simulink model "SMC_control"  (R2025b)
settings: Solver=ode4  StartTime=0.0  StopTime=50  FixedStep=1e-3  RelTol=1e-3
settings Model: Creator=feder  LastModifiedBy=feder

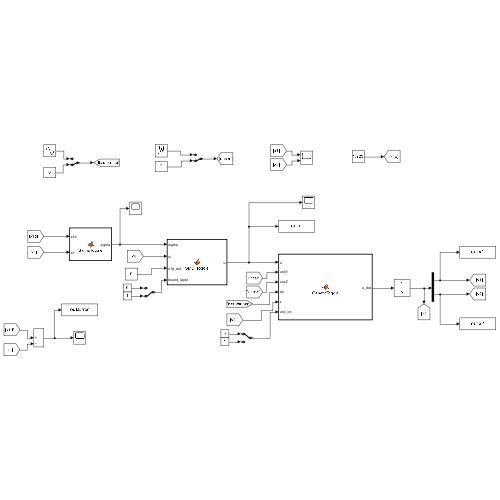
[thumbnail: Simulink's stored preview of the top-level diagram]
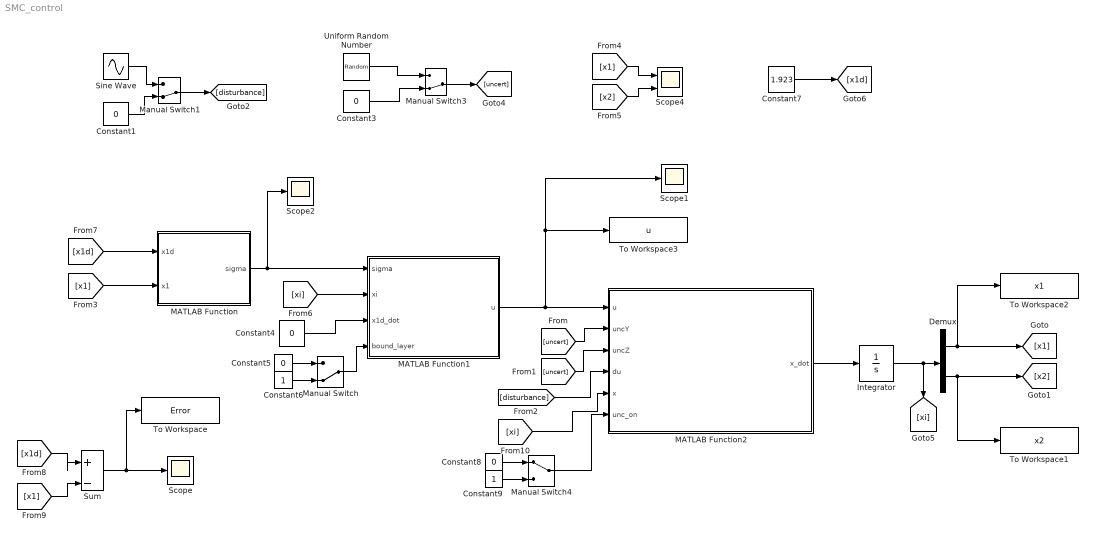
== system SMC_control ==
  Constant{1,3..5,8} (5 alike) : Constant  Value=0
  Constant6 : Constant
  Constant7 : Constant  Value=1.923
  Constant9 : Constant
  Demux : Demux  Outputs=2
  Integrator : Integrator  InitialCondition=[0.127;7.872]
  MATLAB Function : MATLAB Function  TreatAsAtomicUnit=on
  MATLAB Function1 : MATLAB Function  TreatAsAtomicUnit=on
  MATLAB Function2 : MATLAB Function  TreatAsAtomicUnit=on
  Manual Switch : ManualSwitch  CurrentSetting=0
  Manual Switch1 : ManualSwitch  CurrentSetting=0
  Manual Switch3 : ManualSwitch  CurrentSetting=0
  Manual Switch4 : ManualSwitch
  Scope : Scope
      settings: ActiveDisplayYMinimum=-16.327863972090057  ActiveDisplayYMaximum=16.683930684384531
  Scope1 : Scope
      settings: ActiveDisplayYMinimum=-112.46692384419836  ActiveDisplayYMaximum=360.72714778505906
  Scope2 : Scope
      settings: ActiveDisplayYMinimum=-16.118367270297529  ActiveDisplayYMaximum=10.830983390912735  DataLoggingVariableName=ScopeData2
  Scope4 : Scope  NumInputPorts=2
      settings: ActiveDisplayYMinimum=-1.6651704978189028  ActiveDisplayYMaximum=4.1664336792762047  DataLoggingVariableName=ScopeData4
  Sine Wave : Sin  Frequency=2*pi  SampleTime=0
  Sum : Sum  Inputs=|+-
  To Workspace : ToWorkspace  VariableName=Error  SaveFormat=Timeseries  SampleTime=-1
  To Workspace1 : ToWorkspace  VariableName=x2  SaveFormat=Timeseries  SampleTime=-1
  To Workspace2 : ToWorkspace  VariableName=x1  SaveFormat=Timeseries  SampleTime=-1
  To Workspace3 : ToWorkspace  VariableName=u  SaveFormat=Timeseries  SampleTime=-1
  Uniform Random Number : UniformRandomNumber  Minimum=-0.2  Maximum=0.2  SampleTime=1e6  VectorParams1D=off
  wires:
  [x1] -> Scope4/1
  [x2] -> Scope4/2
  Uniform Random Number/1 -> Manual Switch3/1
  Manual Switch3/1 -> [uncert]
  Manual Switch1/1 -> [disturbance]
  Constant3/1 -> Manual Switch3/2
  MATLAB Function/1(sigma) -> Scope2/1, MATLAB Function1/1(sigma)
  [uncert] -> MATLAB Function2/2(uncY)
  [disturbance] -> MATLAB Function2/4(du)
  Constant4/1 -> MATLAB Function1/3(x1d_dot)
  MATLAB Function2/1(x_dot) -> Integrator/1
  Demux/1 -> To Workspace2/1, [x1]
  Demux/2 -> [x2], To Workspace1/1
  Integrator/1 -> Demux/1, [xi]
  [xi] -> MATLAB Function1/2(xi)
  Constant5/1 -> Manual Switch/1
  Constant6/1 -> Manual Switch/2
  Manual Switch/1 -> MATLAB Function1/4(bound_layer)
  Constant7/1 -> [x1d]
  [x1d] -> MATLAB Function/1(x1d)
  [x1d] -> Sum/1
  [x1] -> Sum/2
  Sum/1 -> To Workspace/1, Scope/1
  Constant8/1 -> Manual Switch4/1
  Constant9/1 -> Manual Switch4/2
  Manual Switch4/1 -> MATLAB Function2/6(unc_on)
  [xi] -> MATLAB Function2/5(x)
  MATLAB Function1/1(u) -> MATLAB Function2/1(u), Scope1/1, To Workspace3/1
  [x1] -> MATLAB Function/2(x1)
  Constant1/1 -> Manual Switch1/2
  [uncert] -> MATLAB Function2/3(uncZ)
  Sine Wave/1 -> Manual Switch1/1

== matlab function SMC_control/MATLAB Function1 ==
  data: sigma input; u output; xi input; x1d_dot input; bound_layer input
function u = SMC_Toggle(sigma, xi, x1d_dot, bound_layer)

x1 = xi(1);
x2 = xi(2);

alphaY_nom = 10;     
betaY      = 0.25;
betaZ      = 0.25;


p1      = 9;        % 9 caso nominale
k       = 7;          % 3 caso nominale
epsilon = 0.01;      % 0.5 caso nominale pero va bene anche direttamente 0.01


D  = 1 + betaY/(1 + x2^2) + betaZ/(1 + x1^2);
g1 = 1/((1 + x2^2)*D);                         % first component of g(x)
f1 = alphaY_nom/((1 + x2^2)*D) - x1;           % first component of f(x)


Lie_der_f_sigma = p1*(f1 - x1d_dot);           % L_f sigma + partial_t sigma
Lie_der_g_sigma = p1*g1;                       % L_g sigma


if bound_layer
    if sigma > epsilon
        sw = 1;
    elseif sigma < -epsilon
        sw = -1;
    else
        sw = tanh(sigma/epsilon);              
    end
else
    sw = sign(sigma);
end

u = -(Lie_der_f_sigma + k*sw)/Lie_der_g_sigma;

end

% % ---- Control law (Raw) ----
% u_raw = -(Lie_der_f_sigma + k*sw)/Lie_der_g_sigma;
% 
% % ---- Input Saturation [-10, +30] ----
% % 1. min(u, 30)  -> Se u > 30, diventa 30.
% % 2. max(..., -10) -> Se il risultato è < -10, diventa -10.
% u = max(-10, min(u_raw, 30));
% 
% end

== matlab function SMC_control/MATLAB Function ==
  data: x1d input; x1 input; sigma output
function sigma = SigmaToggle(x1d, x1)
p1 = 9;              
sigma = p1*(x1 - x1d);
end

== matlab function SMC_control/MATLAB Function2 ==
  data: u input; uncY input; uncZ input; du input; x input; x_dot output; unc_on input
function x_dot = GeneticToggle(u, uncY, uncZ, du,x,unc_on)
alphaY_nom = 10;
alphaZ_nom = 10;
betaY_nom  = 0.25;
betaZ_nom  = 0.25;
gammaY     = 1;
gammaZ     = 1;
KY         = 1;
KZ         = 1;
n          = 2;

x1 = x(1);
x2 = x(2);


if unc_on
    alphaY_eff = alphaY_nom*(1 + uncY);
    alphaZ_eff = alphaZ_nom*(1 + uncZ);
    betaY = betaY_nom;  
    betaZ = betaZ_nom;
else
    alphaY_eff = alphaY_nom;
    alphaZ_eff = alphaZ_nom;
    betaY = betaY_nom;
    betaZ = betaZ_nom;
end


u_app = u + du;


alphaY_act = alphaY_eff + u_app;


HZ = 1 / (1 + (x2 / KZ)^n);
HY = 1 / (1 + (x1 / KY)^n);

% Denominator 
D = 1 + betaY*HZ + betaZ*HY;

dx1 = (alphaY_act * HZ / D) - gammaY*x1;
dx2 = (alphaZ_eff * HY / D) - gammaZ*x2;

x_dot = [dx1; dx2];
end
